simulink model "MOSFETBuckSimulinkDevice"  (R2026a)
settings: Solver=ode23t  StopTime=0.05  MaxStep=1e-7  RelTol=1e-4
libraries: fl_lib x6, nesl_utility x3, ee_lib x1, ConverterLibrary x1
Description:
  | Inverted buck converter test for the Simulink MOSFET device: 600 V input, 20 A load current, 100 kHz, 50 % duty, case held at 25 degC.
settings Model: Creator=vsolaise  LastModifiedBy=vsolaise
settings SimscapeCC: SimscapeLogLimitData=off

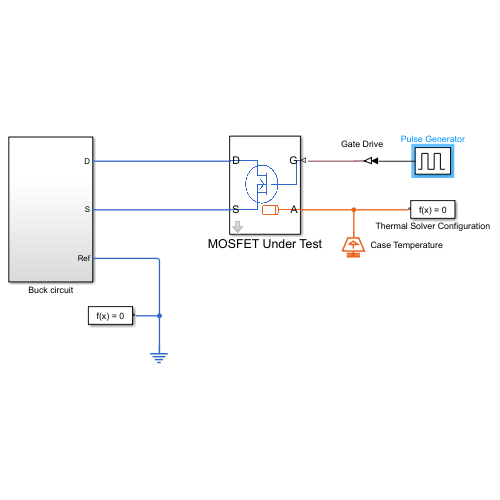
[thumbnail: Simulink's stored preview of the top-level diagram]
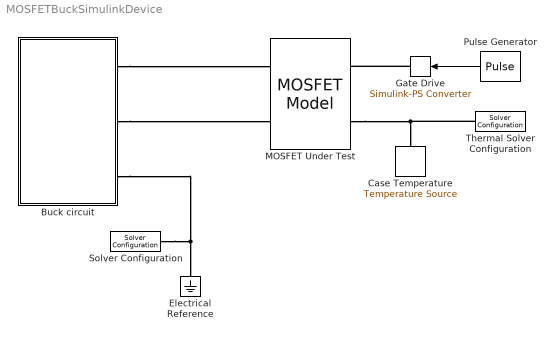
== system MOSFETBuckSimulinkDevice ==
  Buck circuit : Subsystem
  Case Temperature : fl_lib/Thermal/Thermal Sources/Temperature Source  temperature=298.15 K
  Electrical Reference : fl_lib/Electrical/Electrical Elements/Electrical Reference
  Gate Drive : nesl_utility/Simulink-PS Converter  PhysicalDomain=network_engine_domain  SubClassName=ps_input  LeftPortType=input  RightPortType=output  PseudoPeriodic=off  Frequencies=[]  NoiseDistribution=none  NoiseParameters=[]  Unit=1  AffineConversion=off  FilteringAndDerivatives=provide  SimscapeFilterOrder=1  InputFilterTimeConstant=0.001  UdotUserProvided=0
  MOSFET Under Test : ConverterLibrary/Components/MOSFET Model  Vth=3.2 V  Von_data=[-3.075 -1.321 -0.5334 -0.2017 -5.735e-2 0 5.654e-2 0.1988 0.6074 1.756 5.672; -4.404 -1.709 -0.657 -0.2346 -0.0667 0 6.456e-2 0.227 0.6342 1.831 6.194; -4.759 -3.111 -1.191 -0.4253 -0.1209 0 0.1049 0.369 1.1 3.268 12.47; -5.366 -4.667 -1.787 -0.638 -0.1813 0 0.1573 0.5535 1.65 4.902 18.71] V  Tj=[-55 25 150 900] degC  Iout_data=[-99.94 -39.11 -14.94 -5.333 -1.517 0 1.517 5.334 14.94 39.12 99.97] A  Iout_data_loss=[0 16.04 32.08 48.12 64.15 80.19] A  Tj_loss=[-55 25 150 900 1000] degC  Eoff_data=[0 1.079e-4 2.792e-4 6.058e-4 1.107e-3 1.708e-3; 0 1.046e-4 2.706e-4 5.872e-4 1.073e-3 1.655e-3; 0 1.303e-4 3.368e-4 7.31e-4 1.336e-3 2.061e-3; 0 1.433e-4 3.705e-4 8.041e-4 1.47e-3 2.267e-3; 0 1.433e-4 3.705e-4 8.041e-4 1.47e-3 2.267e-3] J  Eon_data=[0 2.53e-4 7.404e-4 1.481e-3 2.418e-3 3.535e-3; 0 2.341e-4 6.85e-4 1.37e-3 2.237e-3 3.27e-3; 0 2.172e-4 6.356e-4 1.272e-3 2.076e-3 3.035e-3; 0 1.955e-4 5.72e-4 1.145e-3 1.868e-3 2.732e-3; 0 1.955e-4 5.72e-4 1.145e-3 1.868e-3 2.732e-3] J  Voff=800 V  Soft_Switching_Flag=on  Tj_diode=[-55 25 150 900 1000] degC  If_data=[0 1.516 5.33 14.93 39.07 99.82] A  Vf_data=[0 3.294 3.769 4.385 5.249 6.672; 0 2.997 3.415 3.921 4.714 5.992; 0 2.624 2.988 3.498 4.274 5.6; 0 2.362 2.689 3.148 3.847 5.04; 0 2.362 2.689 3.148 3.847 5.04] V  thermal_resistance=0.5 K/W  thermal_mass=0.01 J/K  Tj0=25 degC
      settings: SourceProductName=Simscape Power Converter Components
  Pulse Generator : DiscretePulseGenerator  PulseType=Time based  Amplitude=15  Period=1e-05  PulseWidth=50
  Solver Configuration : nesl_utility/Solver Configuration  PhysicalDomain=network_engine_domain  SubClassName=solver  LeftPortType=input  RightPortType=generic  Tones=[]  Harmonics=[]  SimulateNoise=off  Profile=off  UseLocalSampling=off  EnableSwitchedLinearOptims=on  FrequencyDomain=off  UseCCode=off  RelTol=0.001  AbsTol=0.001  MinStep=1e-09  ToWorkspace=off  RevertToSquareIcSolve=off  NumHomotopyIterations=100  PhasorMode=off  PhasorModeNumHarmonics=1  ConsistencySolver=NEWTON_XTOL_AFTER_FTOL  CanonicalOrdering=CANONICAL  OptimizeIntermediates=OPTIMIZED  IndexReductionMethod=DerivativeReplacement  DoDC=off  ResidualTolerance=1e-09  ConsistencyTolSource=GLOBAL  ConsistencyAbsTol=0.001  ConsistencyRelTol=0.001  ConsistencyTolFactor=0.001  UseLocalSolver=off  LocalSolverChoice=NE_BACKWARD_EULER_ADVANCER  ResolveIndetEquations=on  FunctionEvalNumThread=1  LocalSolverSampleTime=0.001  DoFixedCost=off  MaxNonlinIter=3  MaxModeIter=2  ComputeImpulses=off  ImpulseIterations=2  LinearAlgebra=auto  LinearAlgebraNumThread=0  EquationFormulation=NE_TIME_EF  DelaysMemoryBudget=1024  AutomaticFiltering=on  FilteringTimeConstant=0.001  PartitionStorageMethod=AS_NEEDED  PartitionMemoryBudget=1024  PartitionMethod=ROBUST  MultibodyUseLocalSolver=off  MultibodyLocalSolverChoice=ODE1  MultibodyLocalSolverSampleTime=0.001
  Thermal Solver Configuration : nesl_utility/Solver Configuration  PhysicalDomain=network_engine_domain  SubClassName=solver  LeftPortType=input  RightPortType=generic  Tones=[]  Harmonics=[]  SimulateNoise=off  Profile=off  UseLocalSampling=off  EnableSwitchedLinearOptims=on  FrequencyDomain=off  UseCCode=off  RelTol=0.001  AbsTol=0.001  MinStep=1e-09  ToWorkspace=off  RevertToSquareIcSolve=off  NumHomotopyIterations=100  PhasorMode=off  PhasorModeNumHarmonics=1  ConsistencySolver=NEWTON_XTOL_AFTER_FTOL  CanonicalOrdering=CANONICAL  OptimizeIntermediates=OPTIMIZED  IndexReductionMethod=DerivativeReplacement  DoDC=off  ResidualTolerance=1e-09  ConsistencyTolSource=GLOBAL  ConsistencyAbsTol=0.001  ConsistencyRelTol=0.001  ConsistencyTolFactor=0.001  UseLocalSolver=off  LocalSolverChoice=NE_BACKWARD_EULER_ADVANCER  ResolveIndetEquations=on  FunctionEvalNumThread=1  LocalSolverSampleTime=0.001  DoFixedCost=off  MaxNonlinIter=3  MaxModeIter=2  ComputeImpulses=off  ImpulseIterations=2  LinearAlgebra=auto  LinearAlgebraNumThread=0  EquationFormulation=NE_TIME_EF  DelaysMemoryBudget=1024  AutomaticFiltering=on  FilteringTimeConstant=0.001  PartitionStorageMethod=AS_NEEDED  PartitionMemoryBudget=1024  PartitionMethod=ROBUST  MultibodyUseLocalSolver=off  MultibodyLocalSolverChoice=ODE1  MultibodyLocalSolverSampleTime=0.001
  wires:
  Pulse Generator/1 -> Gate Drive/1
  connections:
  Gate Drive/RConn1 -- MOSFET Under Test/LConn1
  Buck circuit/RConn1 -- MOSFET Under Test/RConn1
  Buck circuit/RConn2 -- MOSFET Under Test/RConn2
  MOSFET Under Test/LConn2 -- Thermal Solver Configuration/RConn1 -- Case Temperature/LConn1
  Solver Configuration/RConn1 -- Electrical Reference/LConn1 -- Buck circuit/RConn3

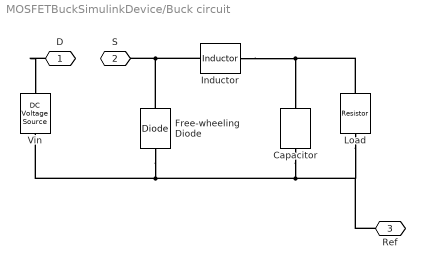
== system MOSFETBuckSimulinkDevice/Buck circuit ==
  Capacitor : fl_lib/Electrical/Electrical Elements/Capacitor  c=2e-05 F  r=1e-6 Ohm  g=0 1/Ohm  i_specify=off  i_priority=None  i=0 A  i_nominal_specify=off  i_nominal_value=1  i_nominal_unit=A  v_specify=off  v_priority=None  v=0 V  v_nominal_specify=off  v_nominal_value=1  v_nominal_unit=V  vc_specify=on  vc_priority=High  vc=300 V  vc_nominal_specify=off  vc_nominal_value=1  vc_nominal_unit=V
  Free-wheeling Diode : ee_lib/Semiconductors & Converters/Diode  ModelType=ee.enum.diode.modelType.pwl  TableType=ee.enum.diode.tableType.IfMat  IfMat=[.07, .12, .19, 1.75, 4.24, 7.32, 11.2; .16, .3, .72, 2.14, 5.02, 8.35, 13.12] A  VfMat=[.9, 1.15, 1.25, 1.5, 1.75, 2.17, 2.6, 2.85; .58, .68, .75, 1.1, 1.38, 1.77, 2.27, 2.7] V  TjVec=[25, 125] degC  VfVec=[.5, .7, .9, 1.3, 1.7, 2.1, 2.5] V  IfVec=[.1, .2, .5, 1, 2, 4, 7, 10] A  IrMat=[1e-06, 2e-06, 5e-06, 1e-05, 2.5e-05, 5e-05, .0001; 2e-06, 5e-06, 1e-05, 4e-05, 8e-05, .0002, .0005] A  VrMat=[10, 100, 200, 250, 300, 325, 350; 10, 70, 160, 220, 270, 300, 320] V  VrVec=[10, 20, 40, 50, 70, 80, 100] V  IrVec=[1e-06, 2e-06, 5e-06, 1e-05, 2e-05, 5e-05, .0001] A  Vf=0.6 V  Ron=0.3 Ohm  Goff=1e-8 S  prmExp=ee.enum.diode.expParam.useTwo  I12=[.0137, .545] A  V12=[.6, .7] V  RS=0 Ohm  Tmeas=298.15 K  IS=1e-12 A  ec=1  I1=0.0137 A  V1=0.6 V  N_series=1  N_parallel=1  ZenerEnable=false  Rz=0.3 Ohm  BV=30 V  C_param=ee.enum.diode.capParam.fixed  CJ=0 pF  CJ0=5 pF  Vvec=[.1, 10, 100] V  Cvec=[3.5, 1, .4] pF  VJ=1 V  Mgrad=0.5  FC=0.5  Q_param=ee.enum.diode.recoveryParam.off  iRM=-7.15 A  iF=4 A  didt=-750 A/us  trr_factor=3  trr=115 ns  Qrr=150 nA*s  Vr=-600 V  Ls=150 nH  Erec=0.03 J  TT=50 ns  tau=100 ns  T_param=ee.enum.diode.temperatureParam.off  Tdevice=298.15 K  I1_T2=0.245 A  V1_T2=0.5 V  IS_T2=1.25e-7 A  Tmeas2=125 degC  XTI_param=ee.enum.diode.xtiParam.pn  XTI=3  EG_param=ee.enum.diode.egapParam.material_si  EG=1.11 eV  dBVdT=0 V/K  enable_fault_input=simscape.enum.onoff.off  i_specify=off  i_priority=None  i=0 A  i_nominal_specify=off  i_nominal_value=1  i_nominal_unit=A  v_specify=off  v_priority=None  v=0 V  v_nominal_specify=off  v_nominal_value=1  v_nominal_unit=V  v_capacitor_specify=off  v_capacitor_priority=None  v_capacitor=0 V  v_capacitor_nominal_specify=off  v_capacitor_nominal_value=1  v_capacitor_nominal_unit=V  Qj_specify=off  Qj_priority=High  Qj=0 C  Qj_nominal_specify=off  Qj_nominal_value=1  Qj_nominal_unit=C  i_diode_specify=off  i_diode_priority=None  i_diode=0 A  i_diode_nominal_specify=off  i_diode_nominal_value=1  i_diode_nominal_unit=A  v_diode_specify=off  v_diode_priority=None  v_diode=0 V  v_diode_nominal_specify=off  v_diode_nominal_value=1  v_diode_nominal_unit=V  i_capacitor_specify=off  i_capacitor_priority=None  i_capacitor=0 A  i_capacitor_nominal_specify=off  i_capacitor_nominal_value=1  i_capacitor_nominal_unit=A  fidelity_level=ee.enum.diode.fidelity.includeChargeDyn  rec_loss_model=ee.enum.diode.reverseRecoveryModelTabulateUpTo3D.fixed  ErecVal=0 J  scaleWithIandV=true  ErecMat=zeros(2, 3) J  ErecMat3D=zeros(2, 3, 2) J  TjrecVec=[298.15, 398.15] K  IfrecVec=[.1, 1, 10] A  IrecVal=10 A  VrecVal=10 V  VrecVec=[0, 100] V  tFilter=1 / 1000 / 100 s  thermal_network_parameterization=ee.enum.thermalNetworkTopology.junctionCase  Rth=[0, 10] K/W  Rth_Cauer=[1, 3, 10] K/W  Rth_Foster=[.08, .14, .22, .16] K/W  thermal_mass_parameterization=ee.enum.thermalNetwork.timeconstant  thermal_mass=[0, 1] J/K  thermal_mass_Cauer=[.1, .3, 1] J/K  thermal_mass_Foster=[.001, .005, .05, .5] J/K  thermal_time_constant=[0, 10] s  thermal_time_constant_Cauer=[1, 3, 10] s  thermal_time_constant_Foster=[7e-05, .0007, .01, .08] s  thermal_mass_initial_temperatures=[25, 25] degC  thermal_mass_initial_temperatures_Cauer=[25, 25, 25] degC  junction_thermal_mass=0.01 J/K  Tvec_initial_Foster=[25, 25, 25, 25] degC  no_thermal_network=0  junction_temperature_specify=off  junction_temperature_priority=None  junction_temperature=25 degC  junction_temperature_nominal_specify=off  junction_temperature_nominal_value=1  junction_temperature_nominal_unit=degC
  Inductor : fl_lib/Electrical/Electrical Elements/Inductor  l=0.00075 H  r=0 Ohm  g=1e-9 1/Ohm  i_specify=off  i_priority=None  i=0 A  i_nominal_specify=off  i_nominal_value=1  i_nominal_unit=A  v_specify=off  v_priority=None  v=0 V  v_nominal_specify=off  v_nominal_value=1  v_nominal_unit=V  i_L_specify=on  i_L_priority=High  i_L=20 A  i_L_nominal_specify=off  i_L_nominal_value=1  i_L_nominal_unit=A
  Load : fl_lib/Electrical/Electrical Elements/Resistor  R=15 Ohm  i_specify=off  i_priority=None  i=0 A  i_nominal_specify=off  i_nominal_value=1  i_nominal_unit=A  v_specify=off  v_priority=None  v=0 V  v_nominal_specify=off  v_nominal_value=1  v_nominal_unit=V
  Vin : fl_lib/Electrical/Electrical Sources/DC Voltage Source  v0=600 V
  D : PMIOPort  Side=Right
  S : PMIOPort  Port=2  Side=Right
  Ref : PMIOPort  Port=3  Side=Right
  connections:
  Free-wheeling Diode/RConn1 -- Inductor/LConn1 -- S/RConn1
  D/RConn1 -- Vin/LConn1
  Inductor/RConn1 -- Load/LConn1 -- Capacitor/LConn1
  Capacitor/RConn1 -- Ref/RConn1 -- Load/RConn1 -- Free-wheeling Diode/LConn1 -- Vin/RConn1
